simulink model "RobotTrajPlatform"  (R2024a)
settings: Solver=ode23t  StartTime=0.0  StopTime=inf  MaxStep=P.Ts  RelTol=1e-3
undefined symbols (not defined in the file): P
libraries: robotmaniplib x3, hdlsllib x1, simulink x1
settings Model: Creator=phoenix_xie  LastModifiedBy=phoenix_xie
settings OptimizationCC: ZeroExternalMemoryAtStartup=off  ZeroInternalMemoryAtStartup=off
settings SFSimCC: SimCustomHeaderCode="#include \"minco_c_api.h\""  SimUserSources=/Users/phoenix_xie/Documents/个人项目/robotics/Minco轨迹规划/minco/minco_c_api.cpp  SimTargetLang=C++
settings SFSimCC: SimUserIncludeDirs=|
  | /Users/phoenix_xie/Documents/个人项目/robotics/Minco轨迹规划/minco
  | /Users/phoenix_xie/Documents/个人项目/robotics/Minco轨迹规划/third_party/GCOPTER/gcopter/include
  | /opt/homebrew/include/eigen3
settings RTWCC: CustomHeaderCode="#include \"minco_c_api.h\""  CustomSource=/Users/phoenix_xie/Documents/个人项目/robotics/Minco轨迹规划/minco/minco_c_api.cpp  TargetLang=C++
settings RTWCC: CustomInclude=|
  | /Users/phoenix_xie/Documents/个人项目/robotics/Minco轨迹规划/minco
  | /Users/phoenix_xie/Documents/个人项目/robotics/Minco轨迹规划/third_party/GCOPTER/gcopter/include
  | /opt/homebrew/include/eigen3
settings GRTTargetCC: TargetLangStandard=C++11 (ISO)  CodeInterfacePackaging=C++ class
settings ExplorerConfigSet: SimMechanicsOpenEditorOnUpdate=off

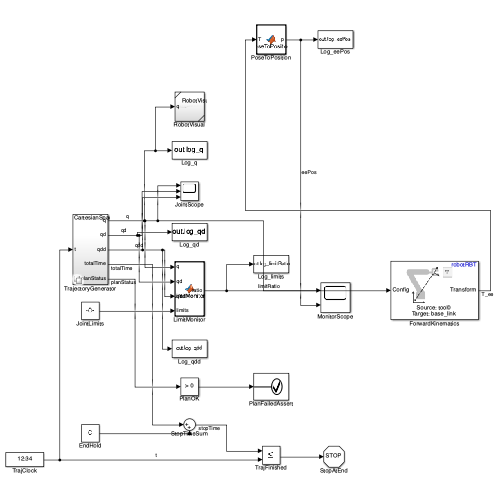
[thumbnail: Simulink's stored preview of the top-level diagram]
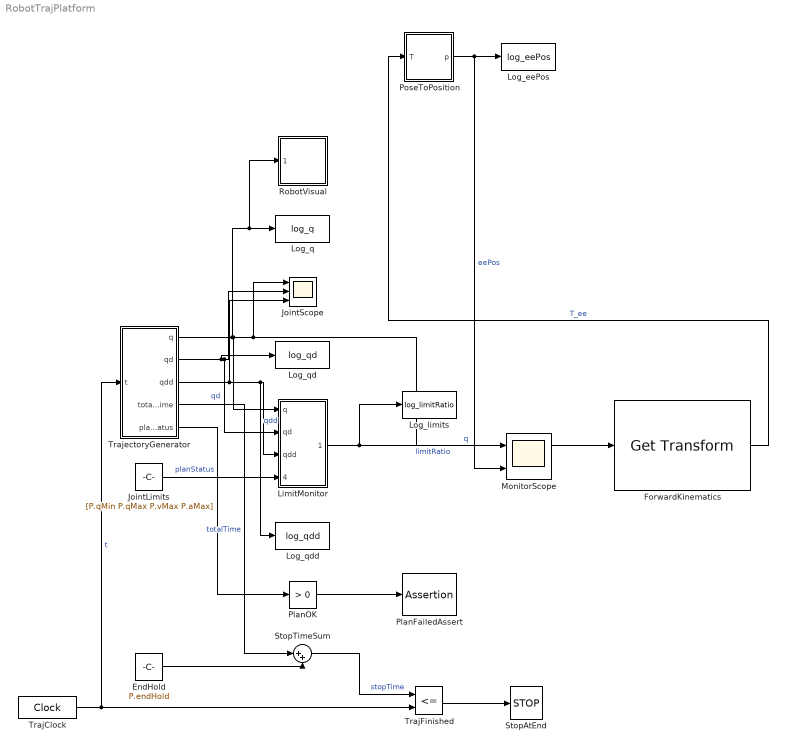
== system RobotTrajPlatform ==
  EndHold : Constant  Value=P.endHold
  ForwardKinematics : robotmaniplib/Get Transform  RigidBodyTree=robotRBT  SourceBody=tool0  TargetBody=base_link  SimulateUsing=Code generation
  JointLimits : Constant  Value=[P.qMin P.qMax P.vMax P.aMax]
  JointScope : Scope  NumInputPorts=3
  LimitMonitor : MATLAB Function  TreatAsAtomicUnit=on
  Log_eePos : ToWorkspace  VariableName=log_eePos  SaveFormat=Timeseries  SampleTime=-1
  Log_limits : ToWorkspace  VariableName=log_limitRatio  SaveFormat=Timeseries  SampleTime=-1
  Log_q : ToWorkspace  VariableName=log_q  SaveFormat=Timeseries  SampleTime=-1
  Log_qd : ToWorkspace  VariableName=log_qd  SaveFormat=Timeseries  SampleTime=-1
  Log_qdd : ToWorkspace  VariableName=log_qdd  SaveFormat=Timeseries  SampleTime=-1
  MonitorScope : Scope  NumInputPorts=2
  PlanFailedAssert : Assertion
  PlanOK : hdlsllib/Logic and Bit Operations/Compare To Zero  relop=>  OutDataTypeStr=boolean
  PoseToPosition : MATLAB Function  TreatAsAtomicUnit=on
  RobotVisual : Subsystem  ReferencedSubsystem=RobotVisual
  StopAtEnd : Stop
  StopTimeSum : Sum  Inputs=|++
  TrajClock : DigitalClock  SampleTime=P.Ts
  TrajFinished : RelationalOperator  Operator=<=
  TrajectoryGenerator : Subsystem  Variant=on
  wires:
  PlanOK/1 -> PlanFailedAssert/1
  TrajectoryGenerator/5(planStatus) -> PlanOK/1  "planStatus"
  TrajFinished/1 -> StopAtEnd/1
  StopTimeSum/1 -> TrajFinished/1  "stopTime"
  EndHold/1 -> StopTimeSum/2
  TrajectoryGenerator/4(totalTime) -> StopTimeSum/1  "totalTime"
  LimitMonitor/1(ratio) -> MonitorScope/1, Log_limits/1  "limitRatio"
  PoseToPosition/1(p) -> MonitorScope/2, Log_eePos/1  "eePos"
  ForwardKinematics/1 -> PoseToPosition/1(T)  "T_ee"
  JointLimits/1 -> LimitMonitor/4(limits)
  TrajectoryGenerator/3(qdd) -> LimitMonitor/3(qdd), Log_qdd/1, JointScope/3  "qdd"
  TrajectoryGenerator/2(qd) -> LimitMonitor/2(qd), JointScope/2, Log_qd/1  "qd"
  TrajectoryGenerator/1(q) -> LimitMonitor/1(q), JointScope/1, ForwardKinematics/1, Log_q/1, RobotVisual/1  "q"
  TrajClock/1 -> TrajFinished/2, TrajectoryGenerator/1(t)  "t"

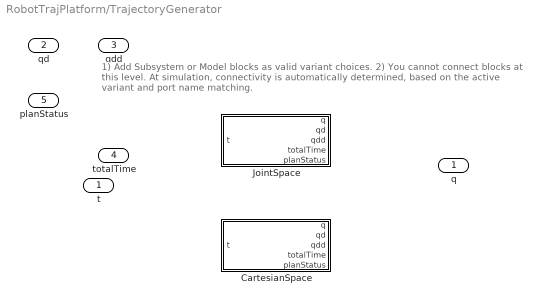
== system RobotTrajPlatform/TrajectoryGenerator ==
  note: 1) Add Subsystem or Model blocks as valid variant choices.
      | 2) You cannot connect blocks at this level. At simulation, connectivity is automatically
      | determined, based on the active variant and port name matching.
  t : Inport
  CartesianSpace : Subsystem  VariantControl=VC_CartesianSpace
  JointSpace : Subsystem  VariantControl=VC_JointSpace
  q : Outport
  qd : Outport  Port=2
  qdd : Outport  Port=3
  totalTime : Outport  Port=4
  planStatus : Outport  Port=5

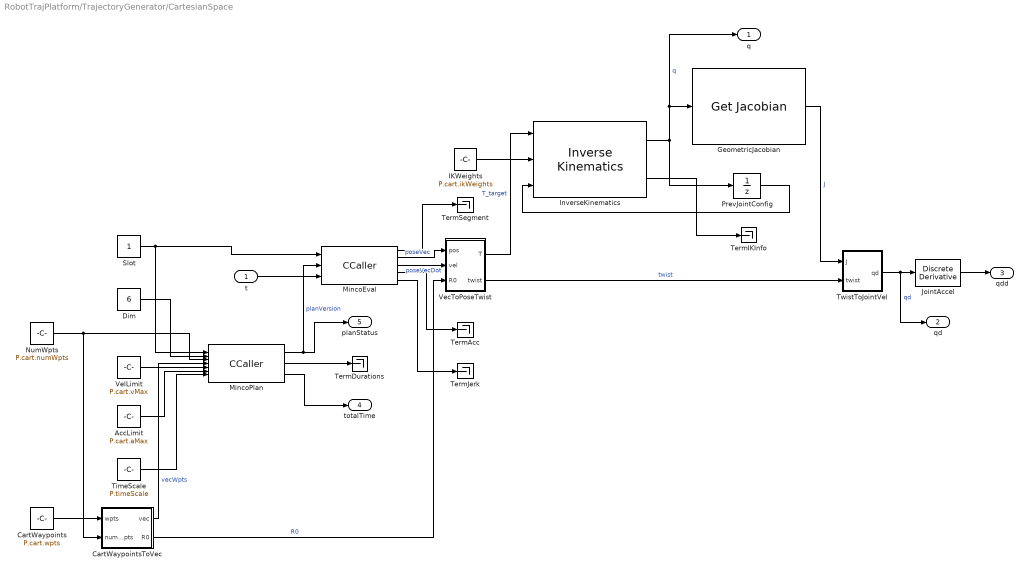
== system RobotTrajPlatform/TrajectoryGenerator/CartesianSpace ==
  t : Inport
  AccLimit : Constant  Value=P.cart.aMax
  CartWaypoints : Constant  Value=P.cart.wpts
  CartWaypointsToVec : MATLAB Function  TreatAsAtomicUnit=on
  Dim : Constant  Value=6  OutDataTypeStr=int32
  GeometricJacobian : robotmaniplib/Get Jacobian  RigidBodyTree=robotRBT  EndEffector=tool0  SimulateUsing=Code generation
  IKWeights : Constant  Value=P.cart.ikWeights
  InverseKinematics : robotmaniplib/Inverse Kinematics  RigidBodyTree=robotRBT  EndEffector=tool0  ShowInfo=on  SolverName=BFGS Gradient Projection  EnforceJointLimits=on  MaxIterations=300  MaxTime=10  GradientTolerance=1e-7  SolutionTolerance=1e-6  StepTolerance=1e-14  ErrorChangeTolerance=1e-12  UseErrorDamping=on  DampingBias=0.0025  SimulateUsing=Code generation
  JointAccel : simulink/Discrete/Discrete Derivative  gainval=1.0  ICPrevScaledInput=0.0  OutMin=[]  OutMax=[]  OutDataType=fixdt(1, 16)  OutScaling=2^-10  DoSatur=off
  MincoEval : CCaller  FunctionName=minco_eval  PortSpecificationStruct="%)30     .    N T   8    (     @         %    \"     @    !     0         %  0 \"0    $    _    07)G3F%M90  4&]R=$YA;64 4V-O<&4     26YD97@     5'EP90      4VEZ90      27-';&]B86P   X    P    !@    @    $          4    (     0    ,    !         !   P!O=70 #@   #     &    \"     0         !0    @    !     P    $         $  # &]U=  .    .     8    (    !          %    \"     $    &     0         0   ...(+4354 chars)"  SampleTime=P.Ts
  MincoPlan : CCaller  FunctionName=minco_plan  PortSpecificationStruct="%)30     .    .!$   8    (     @         %    \"     H    !     0         %  0 \"0    $    _    07)G3F%M90  4&]R=$YA;64 4V-O<&4     26YD97@     5'EP90      4VEZ90      27-';&]B86P   X    P    !@    @    $          4    (     0    ,    !         !   P!O=70 #@   #     &    \"     0         !0    @    !     P    $         $  # &]U=  .    .     8    (    !          %    \"     $    &     0         0   ...(+5564 chars)"  SampleTime=P.Ts
  NumWpts : Constant  Value=P.cart.numWpts  OutDataTypeStr=int32
  PrevJointConfig : UnitDelay  InitialCondition=P.cart.qInit  SampleTime=P.Ts
  Slot : Constant  OutDataTypeStr=int32
  TermAcc : Terminator
  TermDurations : Terminator
  TermIKInfo : Terminator
  TermJerk : Terminator
  TermSegment : Terminator
  TimeScale : Constant  Value=P.timeScale
  TwistToJointVel : MATLAB Function  TreatAsAtomicUnit=on
  VecToPoseTwist : MATLAB Function  TreatAsAtomicUnit=on
  VelLimit : Constant  Value=P.cart.vMax
  q : Outport
  qd : Outport  Port=2
  qdd : Outport  Port=3
  totalTime : Outport  Port=4
  planStatus : Outport  Port=5
  wires:
  InverseKinematics/2 -> TermIKInfo/1
  MincoEval/5 -> TermJerk/1
  MincoEval/4 -> TermAcc/1
  MincoEval/1 -> TermSegment/1
  MincoPlan/2 -> TermDurations/1
  MincoPlan/3 -> totalTime/1
  JointAccel/1 -> qdd/1
  TwistToJointVel/1(qd) -> JointAccel/1, qd/1  "qd"
  VecToPoseTwist/2(twist) -> TwistToJointVel/2(twist)  "twist"
  GeometricJacobian/1 -> TwistToJointVel/1(J)  "J"
  InverseKinematics/1 -> GeometricJacobian/1, q/1, PrevJointConfig/1  "q"
  PrevJointConfig/1 -> InverseKinematics/3
  IKWeights/1 -> InverseKinematics/2
  VecToPoseTwist/1(T) -> InverseKinematics/1  "T_target"
  CartWaypointsToVec/2(R0) -> VecToPoseTwist/3(R0)  "R0"
  MincoEval/3 -> VecToPoseTwist/2(vel)  "poseVecDot"
  MincoEval/2 -> VecToPoseTwist/1(pos)  "poseVec"
  t/1 -> MincoEval/3
  MincoPlan/1 -> planStatus/1, MincoEval/2  "planVersion"
  TimeScale/1 -> MincoPlan/7
  AccLimit/1 -> MincoPlan/6
  VelLimit/1 -> MincoPlan/5
  CartWaypointsToVec/1(vec) -> MincoPlan/4  "vecWpts"
  Dim/1 -> MincoPlan/2
  Slot/1 -> MincoEval/1, MincoPlan/1
  NumWpts/1 -> MincoPlan/3, CartWaypointsToVec/2(numWpts)
  CartWaypoints/1 -> CartWaypointsToVec/1(wpts)

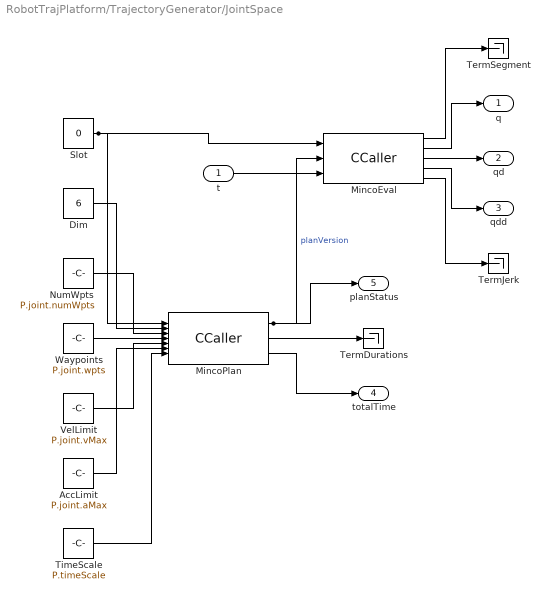
== system RobotTrajPlatform/TrajectoryGenerator/JointSpace ==
  t : Inport
  AccLimit : Constant  Value=P.joint.aMax
  Dim : Constant  Value=6  OutDataTypeStr=int32
  MincoEval : CCaller  FunctionName=minco_eval  PortSpecificationStruct="%)30     .    N T   8    (     @         %    \"     @    !     0         %  0 \"0    $    _    07)G3F%M90  4&]R=$YA;64 4V-O<&4     26YD97@     5'EP90      4VEZ90      27-';&]B86P   X    P    !@    @    $          4    (     0    ,    !         !   P!O=70 #@   #     &    \"     0         !0    @    !     P    $         $  # &]U=  .    .     8    (    !          %    \"     $    &     0         0   ...(+4354 chars)"  SampleTime=P.Ts
  MincoPlan : CCaller  FunctionName=minco_plan  PortSpecificationStruct="%)30     .    .!$   8    (     @         %    \"     H    !     0         %  0 \"0    $    _    07)G3F%M90  4&]R=$YA;64 4V-O<&4     26YD97@     5'EP90      4VEZ90      27-';&]B86P   X    P    !@    @    $          4    (     0    ,    !         !   P!O=70 #@   #     &    \"     0         !0    @    !     P    $         $  # &]U=  .    .     8    (    !          %    \"     $    &     0         0   ...(+5564 chars)"  SampleTime=P.Ts
  NumWpts : Constant  Value=P.joint.numWpts  OutDataTypeStr=int32
  Slot : Constant  Value=0  OutDataTypeStr=int32
  TermDurations : Terminator
  TermJerk : Terminator
  TermSegment : Terminator
  TimeScale : Constant  Value=P.timeScale
  VelLimit : Constant  Value=P.joint.vMax
  Waypoints : Constant  Value=P.joint.wpts
  q : Outport
  qd : Outport  Port=2
  qdd : Outport  Port=3
  totalTime : Outport  Port=4
  planStatus : Outport  Port=5
  wires:
  MincoEval/5 -> TermJerk/1
  MincoEval/1 -> TermSegment/1
  MincoPlan/2 -> TermDurations/1
  MincoPlan/3 -> totalTime/1
  MincoEval/4 -> qdd/1
  MincoEval/3 -> qd/1
  MincoEval/2 -> q/1
  t/1 -> MincoEval/3
  MincoPlan/1 -> planStatus/1, MincoEval/2  "planVersion"
  TimeScale/1 -> MincoPlan/7
  AccLimit/1 -> MincoPlan/6
  VelLimit/1 -> MincoPlan/5
  Waypoints/1 -> MincoPlan/4
  NumWpts/1 -> MincoPlan/3
  Dim/1 -> MincoPlan/2
  Slot/1 -> MincoEval/1, MincoPlan/1

== matlab function RobotTrajPlatform/LimitMonitor ==
  data: q input; ratio output; qd input; qdd input; limits input
function ratio = LimitMonitor(q, qd, qdd, limits)
%#codegen
% limits = [qMin qMax vMax aMax]，每行一个关节
% ratio  = [max|qd|/vMax; max|qdd|/aMax; 关节越限标志]
ratio = [max(abs(qd) ./ limits(:, 3)); ...
         max(abs(qdd) ./ limits(:, 4)); ...
         double(any(q < limits(:, 1) | q > limits(:, 2)))];

== matlab function RobotTrajPlatform/PoseToPosition ==
  data: T input; p output
function p = PoseToPosition(T)
%#codegen
p = T(1:3, 4);

== matlab function RobotTrajPlatform/TrajectoryGenerator/CartesianSpace/CartWaypointsToVec ==
  data: wpts input; vec output; numWpts input; R0 output
function [vec, R0] = CartWaypointsToVec(wpts, numWpts)
%#codegen
% wpts 每列 [x y z yaw pitch roll]（ZYX 欧拉角）。姿态转成相对首个路径点的旋转向量 w_k，
% 满足 R_k = R0 * Exp(w_k)，从而可以与位置一起用 MINCO 规划。各路径点姿态须在首点 180 度以内。
vec = zeros(size(wpts));
R0 = eulZYX(wpts(4:6, 1));
for k = 1:double(numWpts)
    vec(1:3, k) = wpts(1:3, k);
    vec(4:6, k) = so3Log(R0' * eulZYX(wpts(4:6, k)));
end
end

function R = eulZYX(e)
cz = cos(e(1)); sz = sin(e(1)); cy = cos(e(2)); sy = sin(e(2)); cx = cos(e(3)); sx = sin(e(3));
R = [cz -sz 0; sz cz 0; 0 0 1] * [cy 0 sy; 0 1 0; -sy 0 cy] * [1 0 0; 0 cx -sx; 0 sx cx];
end

function w = so3Log(R)
th = acos(min(max((trace(R) - 1) / 2, -1), 1));
v = [R(3,2) - R(2,3); R(1,3) - R(3,1); R(2,1) - R(1,2)];
if th < 1e-9
    w = 0.5 * v;
elseif pi - th < 1e-6
    [~, i] = max(diag(R));
    a = R(:, i); a(i) = a(i) + 1;
    w = th * a / norm(a);
else
    w = th / (2 * sin(th)) * v;
end
end

== matlab function RobotTrajPlatform/TrajectoryGenerator/CartesianSpace/VecToPoseTwist ==
  data: pos input; T output; vel input; R0 input; twist output
function [T, twist] = VecToPoseTwist(pos, vel, R0)
%#codegen
% pos/vel = [p; w] 及其导数。R = R0*Exp(w)，基座系角速度 omega = R0*Jl(w)*dw。
% twist = [omega; v]，与 Get Jacobian 的行顺序一致。
w = pos(4:6);
th = norm(w);
W = [0 -w(3) w(2); w(3) 0 -w(1); -w(2) w(1) 0];
if th < 1e-9
    E = eye(3) + W;
    Jl = eye(3) + 0.5 * W;
else
    E = eye(3) + sin(th) / th * W + (1 - cos(th)) / th^2 * (W * W);
    Jl = eye(3) + (1 - cos(th)) / th^2 * W + (th - sin(th)) / th^3 * (W * W);
end
T = [R0 * E, pos(1:3); 0 0 0 1];
twist = [R0 * Jl * vel(4:6); vel(1:3)];
end

== matlab function RobotTrajPlatform/TrajectoryGenerator/CartesianSpace/TwistToJointVel ==
  data: J input; qd output; twist input
function qd = TwistToJointVel(J, twist)
%#codegen
% 阻尼最小二乘伪逆，奇异位姿附近保持数值稳定
lambda = 1e-3;
qd = J' * ((J * J' + lambda^2 * eye(6)) \ twist(:));
end
